simulink library "full_bridge_three_level_ttype_igbt_based_model"  (R2025b)
settings: Solver=VariableStepAuto  StartTime=0.0  StopTime=10.0  RelTol=1e-3
undefined symbols (not defined in the file): tc
libraries: fl_lib x80, nesl_utility x48, ee_lib x8
(part 3 of 3)

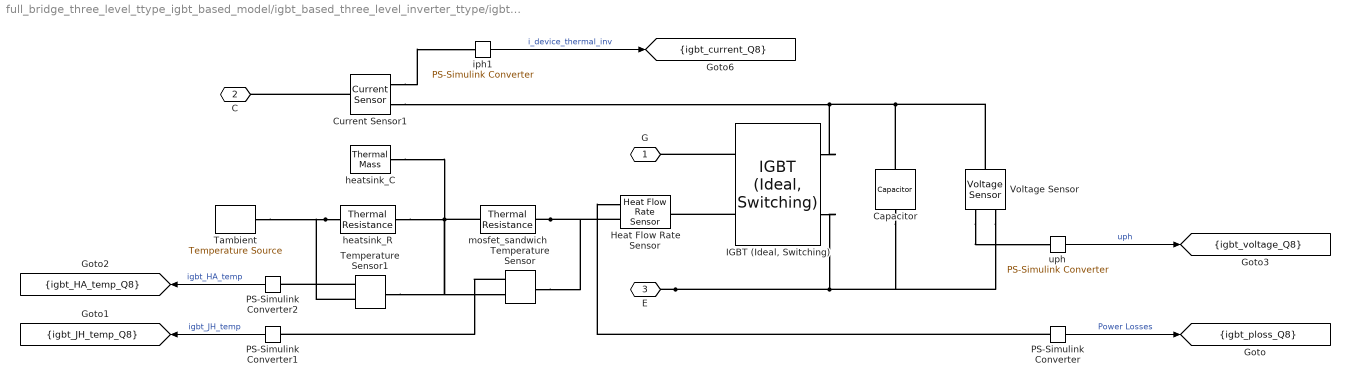
== system full_bridge_three_level_ttype_igbt_based_model/igbt_based_three_level_inverter_ttype/igbt_thermal_8 ==
  Capacitor : fl_lib/Electrical/Electrical Elements/Capacitor  c=Csnubber F  r=Rsnubber Ohm  g=0 1/Ohm  i_specify=off  i_priority=None  i=0 A  i_nominal_specify=off  i_nominal_value=1  i_nominal_unit=A  v_specify=off  v_priority=None  v=0 V  v_nominal_specify=off  v_nominal_value=1  v_nominal_unit=V  vc_specify=off  vc_priority=High  vc=0 V  vc_nominal_specify=off  vc_nominal_value=1  vc_nominal_unit=V
  Current Sensor1 : fl_lib/Electrical/Electrical Sensors/Current Sensor
  Heat Flow Rate Sensor : fl_lib/Thermal/Thermal Sensors/Heat Flow Rate Sensor
  "IGBT (Ideal, Switching)" : ee_lib/Semiconductors & Converters/IGBT (Ideal, Switching)  port_option=ee.enum.controlport.ps  Vf=Vce_sat_inv V  Ron=Rce_on_inv Ohm  Goff=1e-5 1/Ohm  Vth=Vth_inv V  diode_param=ee.enum.semiconductors.protectionDiode.nodynamics  diode_Vf=Vdon_diode_inv V  diode_Ron=Rdon_diode_inv Ohm  diode_Goff=1e-5 1/Ohm  diode_C=50e-9 F  diode_iRM=-235 A  diode_iF=300 A  diode_idot=-50 A/us  diode_trr_param=ee.enum.converters.diodeReverseParam.trr_factor  diode_trr_factor=3  diode_trr=15 us  diode_Qrr=1500 s*uA  ice_specify=off  ice_priority=None  ice=0 A  ice_nominal_specify=off  ice_nominal_value=1  ice_nominal_unit=A  vce_specify=off  vce_priority=None  vce=0 V  vce_nominal_specify=off  vce_nominal_value=1  vce_nominal_unit=V  vge_specify=off  vge_priority=None  vge=0 V  vge_nominal_specify=off  vge_nominal_value=1  vge_nominal_unit=V  thermal_loss_option=ee.enum.converters.thermalLossOption.constantvalues  Von_data=[0, .1, .6, .8, 1, 1.3, 1.6, 2, 2.4; 0, .1, .7, 1, 1.2, 1.5, 1.9, 2.4, 2.8] V  Tj=[298.15, 398.15] K  Iout_data=[0, .1, 1, 5, 10, 20, 40, 70, 100] A  Eon_data=[0, .0024, .024, .12, .2, .48, 1.04, 2.16, 3.24; 0, .003, .03, .15, .25, .6, 1.3, 2.7, 4.05] * 1e-3 J  Eoff_data=[0, .0007, .0066, .033, .066, .17, .33, .83, 1.5; 0, .001, .01, .05, .1, .25, .5, 1.2, 2.2] * 1e-3 J  Eon_data_3D=[zeros(2, 9, 3)] J  Eoff_data_3D=[zeros(2, 9, 3)] J  Tj_loss=[298.15, 398.15] K  Iout_data_loss=[0, .1, 1, 5, 10, 20, 40, 70, 100] A  tabulateWithVce=false  Vce_loss=[0, 150, 300] V  Eon_scalar=Eon_inv J  Eoff_scalar=Eoff_inv J  Voff=Voff_sw_loss_inv V  Iout_scalar=Ion_sw_loss_inv A  useCurrentFromPreviousCycle=true  useVoltageFromPreviousCycle=true  diodeModelType=ee.enum.converters.diodeModelType.pwl  diodeTableType=ee.enum.diode.tableType.IfMat  diode_ReverseIVType=ee.enum.diode.diodeReverseIV.constant  diode_IfMat=[.07, .12, .19, 1.75, 4.24, 7.32, 11.2; .16, .3, .72, 2.14, 4.02, 6.35, 9.12] A  diode_VfMat=[.9, 1.15, 1.25, 1.5, 1.75, 2.17, 2.6, 2.85; .58, .68, .75, 1.1, 1.38, 1.77, 2.27, 2.7] V  diode_TjVec=[25, 125] degC  diode_VfVec=[.5, .7, .9, 1.3, 1.7, 2.1, 2.5] V  diode_IfVec=[.1, .2, .5, 1, 2, 4, 7, 10] A  diode_IrMat=[1e-06, 2e-06, 5e-06, 1e-05, 2.5e-05, 5e-05, .0001; 2e-06, 5e-06, 1e-05, 4e-05, 8e-05, .0002, .0005] A  diode_VrMat=[10, 100, 200, 250, 300, 325, 350; 10, 70, 160, 220, 270, 300, 320] V  diode_VrVec=[10, 20, 40, 50, 70, 80, 100] V  diode_IrVec=[1e-06, 2e-06, 5e-06, 1e-05, 2e-05, 5e-05, .0001] A  diode_Vr=-600 V  diode_Ls=150 nH  diode_Erec=0.03 J  diode_rec_loss_model=ee.enum.diode.reverseRecoveryModel.fixed  diode_ErecVal=Erec_inv J  diode_scaleWithIandV=true  diode_ErecMat=zeros(2, 3) J  diode_TjrecVec=[298.15, 398.15] K  diode_IfrecVec=[.1, 1, 10] A  diode_IrecVal=Ion_sw_loss_inv A  diode_VrecVal=Voff_sw_loss_inv V  diode_tFilter=tc s  separateThermalPortForDiode=false  thermal_network_parameterization=ee.enum.thermalNetworkTopology.external  Rth=[.08, .5] K/W  Rth_Cauer=[.08, .1, .5] K/W  Rth_Foster=[.08, .14, .22, .16] K/W  thermal_mass_parameterization=ee.enum.thermalNetwork.timeconstant  thermal_mass=[.01, .5] J/K  thermal_mass_Cauer=[.01, .1, .5] J/K  thermal_mass_Foster=[.001, .005, .05, .5] J/K  thermal_time_constant=[.001, .2] s  thermal_time_constant_Cauer=[.001, .1, .2] s  thermal_time_constant_Foster=[7e-05, .0007, .01, .08] s  thermal_mass_initial_temperatures=[25, 25] degC  thermal_mass_initial_temperatures_Cauer=[25, 25, 25] degC  junction_thermal_mass=JunctionTermalMass J/K  Tvec_initial_Foster=[25, 25, 25, 25] degC  RthDiode=[.03, .2] K/W  RthCauerDiode=[.03, .1, .2] K/W  RthFosterDiode=[.03, .2] K/W  thermalMassDiode=[3, 25] J/K  thermalMassCauerDiode=[3, 10, 25] J/K  thermalMassFosterDiode=[33, 50] J/K  thermalTauDiode=[.1, 5] s  thermalTauCauerDiode=[.1, 1, 5] s  thermalTauFosterDiode=[1, 10] s  thermalMassInitTempDiode=[25, 25] degC  thermalMassInitTempCauerDiode=[25, 25, 25] degC  junctionthermalMassDiode=0.1 J/K  TVecInitialFosterDiode=[25, 25, 25, 25] degC  no_thermal_network=0  IGBT_junction_temperature_specify=on  IGBT_junction_temperature_priority=High  IGBT_junction_temperature=Tambient degC  IGBT_junction_temperature_nominal_specify=off  IGBT_junction_temperature_nominal_value=1  IGBT_junction_temperature_nominal_unit=degC  diode_junction_temperature_specify=off  diode_junction_temperature_priority=None  diode_junction_temperature=25 degC  diode_junction_temperature_nominal_specify=off  diode_junction_temperature_nominal_value=1  diode_junction_temperature_nominal_unit=degC  Qj_specify=off  Qj_priority=None  Qj=0 W  Qj_nominal_specify=off  Qj_nominal_value=1  Qj_nominal_unit=W  accumulatedSwitchingLosses_specify=off  accumulatedSwitchingLosses_priority=None  accumulatedSwitchingLosses=0 J
      settings: InternalSimscapePortConfiguration="{\"Bottom\":[],\"Left\":[{\"id\":\"G\",\"label\":\"\",\"type\":\"input\"},{\"id\":\"H\",\"label\":\"\",\"type\":\"foundation.thermal.thermal\"}],\"Right\":[{\"id\":\"C\",\"label\":\"\",\"type\":\"foundation.electrical.electrical\"},{\"id\":\"E\",\"label\":\"\",\"type\":\"foundation.electrical.electrical\"}],\"Top\":[]}"
  PS-Simulink Converter : nesl_utility/PS-Simulink Converter  PhysicalDomain=network_engine_domain  SubClassName=ps_output  LeftPortType=input  RightPortType=output  PseudoPeriodic=off  Frequencies=[]  VectorFormat=1-D array  Unit=W  AffineConversion=off
  PS-Simulink Converter1 : nesl_utility/PS-Simulink Converter  PhysicalDomain=network_engine_domain  SubClassName=ps_output  LeftPortType=input  RightPortType=output  PseudoPeriodic=off  Frequencies=[]  VectorFormat=1-D array  Unit=degC  AffineConversion=off
  PS-Simulink Converter2 : nesl_utility/PS-Simulink Converter  PhysicalDomain=network_engine_domain  SubClassName=ps_output  LeftPortType=input  RightPortType=output  PseudoPeriodic=off  Frequencies=[]  VectorFormat=1-D array  Unit=degC  AffineConversion=off
  Tambient : fl_lib/Thermal/Thermal Sources/Temperature Source  temperature=Tambient degC
  Temperature Sensor : fl_lib/Thermal/Thermal Sensors/Temperature Sensor  temperature_measure=foundation.enum.MeasurementReference.difference
  Temperature Sensor1 : fl_lib/Thermal/Thermal Sensors/Temperature Sensor  temperature_measure=foundation.enum.MeasurementReference.difference
  Voltage Sensor : fl_lib/Electrical/Electrical Sensors/Voltage Sensor
  heatsink_C : fl_lib/Thermal/Thermal Elements/Thermal Mass  mass_type=foundation.enum.constant_variable.constant  mass=mass_heatsink kg  sp_heat=specific_heat J/(K*kg)  mass_min=1e-6 kg  num_ports=foundation.enum.numPorts2.one  m_specify=off  m_priority=High  m=1 kg  m_nominal_specify=off  m_nominal_value=1  m_nominal_unit=kg  T_specify=on  T_priority=High  T=DThs_init+Tambient degC  T_nominal_specify=off  T_nominal_value=1  T_nominal_unit=K  Q_specify=off  Q_priority=High  Q=0 W  Q_nominal_specify=off  Q_nominal_value=1  Q_nominal_unit=W
  heatsink_R : fl_lib/Thermal/Thermal Elements/Thermal Resistance  resistance=rth_mosfet_HA_inv K/W  T_specify=off  T_priority=High  T=0 deltadegC  T_nominal_specify=off  T_nominal_value=1  T_nominal_unit=K  Q_specify=off  Q_priority=None  Q=0 W  Q_nominal_specify=off  Q_nominal_value=1  Q_nominal_unit=W
  iph1 : nesl_utility/PS-Simulink Converter  PhysicalDomain=network_engine_domain  SubClassName=ps_output  LeftPortType=input  RightPortType=output  PseudoPeriodic=off  Frequencies=[]  VectorFormat=1-D array  Unit=A  AffineConversion=off
  mosfet_sandwich : fl_lib/Thermal/Thermal Elements/Thermal Resistance  resistance=rth_mosfet_JH_inv K/W  T_specify=off  T_priority=High  T=0 degC  T_nominal_specify=off  T_nominal_value=1  T_nominal_unit=K  Q_specify=off  Q_priority=None  Q=0 W  Q_nominal_specify=off  Q_nominal_value=1  Q_nominal_unit=W
  uph : nesl_utility/PS-Simulink Converter  PhysicalDomain=network_engine_domain  SubClassName=ps_output  LeftPortType=input  RightPortType=output  PseudoPeriodic=off  Frequencies=[]  VectorFormat=1-D array  Unit=V  AffineConversion=off
  G : PMIOPort  Side=Left
  C : PMIOPort  Port=2  Side=Left
  E : PMIOPort  Port=3  Side=Right
  tag scope: igbt_HA_temp_Q8=scoped, igbt_JH_temp_Q8=scoped, igbt_current_Q8=scoped, igbt_ploss_Q8=scoped, igbt_voltage_Q8=scoped
  wires:
  uph/1 -> [igbt_voltage_Q8]  "uph"
  iph1/1 -> [igbt_current_Q8]  "i_device_thermal_inv"
  PS-Simulink Converter1/1 -> [igbt_JH_temp_Q8]  "igbt_JH_temp"
  PS-Simulink Converter2/1 -> [igbt_HA_temp_Q8]  "igbt_HA_temp"
  PS-Simulink Converter/1 -> [igbt_ploss_Q8]  "Power Losses"
  connections:
  Voltage Sensor/RConn1 -- uph/LConn1
  Current Sensor1/RConn1 -- iph1/LConn1
  Voltage Sensor/LConn1 -- Capacitor/LConn1 -- "IGBT (Ideal, Switching)"/RConn1 -- Current Sensor1/RConn2
  Current Sensor1/LConn1 -- C/RConn1
  "IGBT (Ideal, Switching)"/LConn2 -- Heat Flow Rate Sensor/LConn1
  Temperature Sensor1/RConn2 -- PS-Simulink Converter2/LConn1
  heatsink_R/RConn1 -- Temperature Sensor1/RConn1 -- Tambient/LConn1
  Temperature Sensor/RConn2 -- PS-Simulink Converter1/LConn1
  heatsink_C/LConn1 -- heatsink_R/LConn1 -- Temperature Sensor/RConn1 -- Temperature Sensor1/LConn1 -- mosfet_sandwich/RConn1
  mosfet_sandwich/LConn1 -- Heat Flow Rate Sensor/RConn2 -- Temperature Sensor/LConn1
  PS-Simulink Converter/LConn1 -- Heat Flow Rate Sensor/RConn1
  "IGBT (Ideal, Switching)"/LConn1 -- G/RConn1
  E/RConn1 -- Capacitor/RConn1 -- Voltage Sensor/RConn2 -- "IGBT (Ideal, Switching)"/RConn2
